simulink model "P480HZ"  (Simulink 7.5)
settings: Solver=FixedStepDiscrete  StartTime=0.0  StopTime=10.0  FixedStep=0.00008  RelTol=1e-3
libraries: dsPICdrivers x2
settings Model: Creator=Thierry  LastModifiedBy=Thierry
settings OptimizationCC: OptimizeModelRefInitCode=on  LifeSpan=1
settings HardwareCC: ProdBitPerInt=16  ProdEndianess=LittleEndian  ProdWordSize=16  ProdHWDeviceType=16-bit Generic
settings RTWCC: SystemTargetFile=dspic.tlc  TemplateMakefile=dspic_pic30_gcc.tmf  PostCodeGenCommand=dsPIC_Compile()  Description=Embedded Target for Microchip dsPIC (real-time)  ProcessScript=dspic_make_rtw_hook
settings CodeAppCC: IgnoreCustomStorageClasses=off
settings STFCustomTargetCC: ModelReferenceCompliant=off  IncludeMdlTerminateFcn=off  CombineOutputUpdateFcns=on  SuppressErrorStatus=on  ERTCustomFileBanners=on  SupportContinuousTime=off  SupportNonInlinedSFcns=off  SystemTargetFile=dspic.tlc
settings ERTTargetCC: MultiwordLength=2048  ModelReferenceCompliant=off  ParMdlRefBuildCompliant=off  CompOptLevelCompliant=off  IncludeMdlTerminateFcn=off  SuppressErrorStatus=on  ERTFirstTimeCompliant=off  ModelStepFunctionPrototypeControlCompliant=off  CPPClassGenCompliant=off  ExtModeMexFile=noextcomm  InlinedParameterPlacement=NonHierarchical  ERTSrcFileBannerTemplate=dsPIC_code_template.cgt  ERTHdrFileBannerTemplate=dsPIC_code_template.cgt  ERTDataSrcFileTemplate=dsPIC_code_template.cgt  ERTDataHdrFileTemplate=dsPIC_code_template.cgt  ERTCustomFileTemplate=dsPIC_main.tlc  ConvertIfToSwitch=off
settings CustomProperty: DataType=string  Value=C:\PROGRA~1\MATLAB\R2010a\bin\win32\gmake

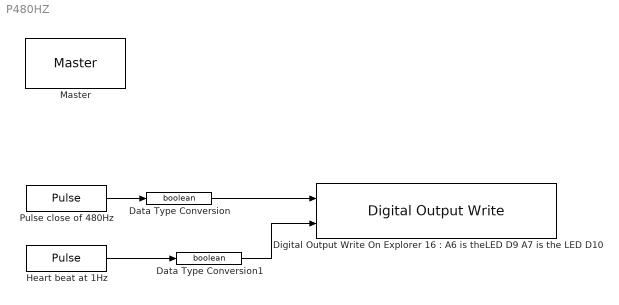
== system P480HZ ==
  Data Type Conversion : DataTypeConversion  OutDataTypeMode=boolean  OutDataType=fixdt(1, 16)  OutScaling=2^0  OutDataTypeStr=boolean
  Data Type Conversion1 : DataTypeConversion  OutDataTypeMode=boolean  OutDataType=fixdt(1, 16)  OutScaling=2^0  OutDataTypeStr=boolean
  "Digital Output Write On Explorer 16 : A6 is theLED D9 A7 is the LED D10" : dsPICdrivers/Digital I//O/Digital Output Write  Tag=dsPIC_Digital_Output  Priority=5  PORT=A  Pin=[6 7]  Simultaneous=off  OrderingInOutPopup=None
  Heart beat at 1Hz : DiscretePulseGenerator  PulseType=Time based  Amplitude=1  Period=1  PulseWidth=50  PhaseDelay=0  SampleTime=0.00008
  Master : dsPICdrivers/Master  Tag=dsPIC_MASTER  Priority=1  TimeStepType=Timer1  picType=33fJ256GP710  fcy=40000000  Quartz_33f=8e6  PLLActive_33f=on  fcyDesired_33f=40000000  tmr1="[1  3199  1.4211e-014]"  tmr1Info="Time Step : 8e-005  ;   Error : 1.4211e-014%  PR1=3199"  tmr2345="[0  0  0  0  0  0  0  0]"  tmr2345cfg=[-1 -1 -1 -1 -1 -1 -1 -1]  IOautoConf=on  typePort="[ 0   0   0   0   0   0  10  10   0   0   0   0   0   0   0   0   0   0   0   0   0   0   0   0   0   0   0   0   0   0   0   0   0   0   0   0   0   0   0   0   0   0   0   0   0   0   0   0   0   0   0   0   0   0   0   0   0   0   0   0   0   0   0   0   0   0   0   0   0   0   0   0   0   0   0   0   0   0   0   0   0   0   0   0   0   0   0   0   0   0   0   0   0   0   0   0   0   0   0   0   0   0   0   0   0   0   0   0   0   0   0   0 ]"  TRIS="[ 65343  65535  65535  65535  65535  65535  65535 ]"  ADPCFG=12582912  MasterBusyPort=None  MasterOverloadPort=None  FOSC=Quartz (XT - HS)  ClockSwitchMonitor=Both disabled  TempProtection_33f=TEMP_ON  FPBOR=<empty>  PWRT=disable  MCLR=<empty>  ICD=ICS_NONE  JTAGEN=JTAGEN_OFF  PowerSave=off  OverrideFcy=off  NewFcy=1e6  PR2345="[65535  65535  65535  65535  65535  65535  65535  65535]"
  Pulse close of 480Hz : DiscretePulseGenerator  Amplitude=1  Period=26  PulseWidth=13  PhaseDelay=0  SampleTime=0.00008
  wires:
  Pulse close of 480Hz/1 -> Data Type Conversion/1
  Data Type Conversion/1 -> "Digital Output Write On Explorer 16 : A6 is theLED D9 A7 is the LED D10"/1
  Heart beat at 1Hz/1 -> Data Type Conversion1/1
  Data Type Conversion1/1 -> "Digital Output Write On Explorer 16 : A6 is theLED D9 A7 is the LED D10"/2
